simulink model "chaine_qpsk"  (R2023b)
settings: Solver=FixedStepDiscrete  StartTime=0.0  StopTime=(N/2 - 1)*2*Tb  FixedStep=2*Tb  RelTol=1e-3
values from neighbouring files (symbols this model uses):
  graine = P.graine    [parametres.m]    (also in parametres_perso.m = mod(sum(c .* (1:numel(c)) * 31) + 7 * numel(c), 2^31 - 1); partie2_1.m)
  N0 = Es / (2*g)    (= 0.158113883008)    [creer_qpsk.m]    (also in creer_qpsk_hamming.m = 0.276699295265; parametres.m = Eb / 10^(EbN0dB/10))
  Tb = 1    [parametres.m]    (also in partie2_1.m)
libraries: simulink x3
settings Model: Creator=e2507477  LastModifiedBy=e2507477

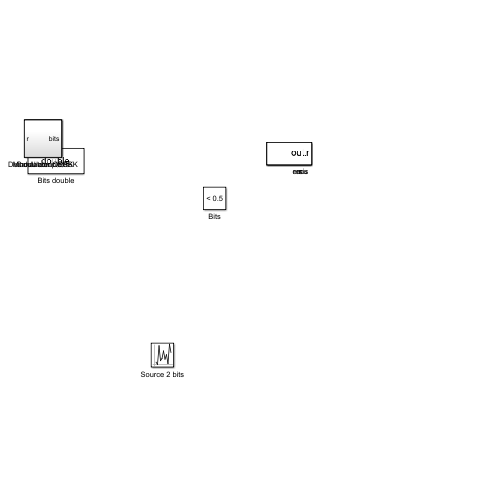
[thumbnail: Simulink's stored preview of the top-level diagram]
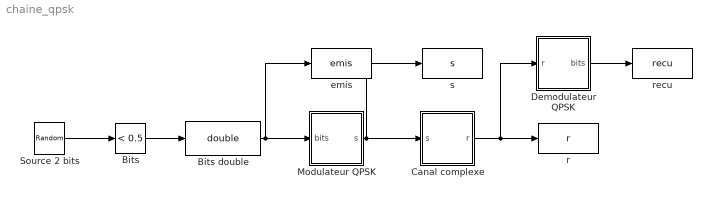
== system chaine_qpsk ==
  Bits : simulink/Logic and Bit Operations/Compare To Constant  relop=<  const=0.5  OutDataTypeStr=boolean
  Bits double : DataTypeConversion  OutDataTypeStr=double  SaturateOnIntegerOverflow=off  RndMeth=Floor
  Canal complexe : Subsystem
  Demodulateur QPSK : Subsystem
  Modulateur QPSK : Subsystem
  Source 2 bits : UniformRandomNumber  Minimum=zeros(1,2)  Maximum=ones(1,2)  Seed=round(graine) + 7919*(0:1)  SampleTime=2*Tb
  emis : ToWorkspace  VariableName=emis  SampleTime=-1
  r : ToWorkspace  VariableName=r  SampleTime=-1
  recu : ToWorkspace  VariableName=recu  SampleTime=-1
  s : ToWorkspace  VariableName=s  SampleTime=-1
  wires:
  Source 2 bits/1 -> Bits/1
  Bits/1 -> Bits double/1
  Bits double/1 -> Modulateur QPSK/1(bits), emis/1
  Modulateur QPSK/1(s) -> Canal complexe/1(s), s/1
  Canal complexe/1(r) -> Demodulateur QPSK/1(r), r/1
  Demodulateur QPSK/1(bits) -> recu/1

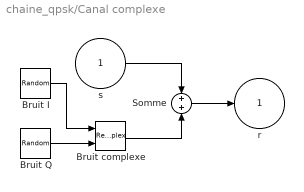
== system chaine_qpsk/Canal complexe ==
  s : Inport
  Bruit I : RandomNumber  Variance=N0/2  Seed=round(graine) + 50000  SampleTime=2*Tb
  Bruit Q : RandomNumber  Variance=N0/2  Seed=round(graine) + 60000  SampleTime=2*Tb
  Bruit complexe : RealImagToComplex
  Somme : Sum
  r : Outport
  wires:
  Somme/1 -> r/1
  Bruit complexe/1 -> Somme/2
  Bruit Q/1 -> Bruit complexe/2
  Bruit I/1 -> Bruit complexe/1
  s/1 -> Somme/1

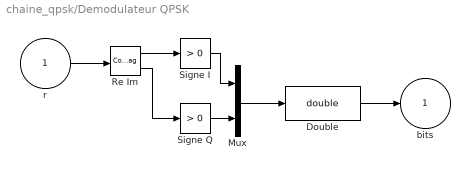
== system chaine_qpsk/Demodulateur QPSK ==
  r : Inport
  Double : DataTypeConversion  OutDataTypeStr=double  SaturateOnIntegerOverflow=off  RndMeth=Floor
  Mux : Mux  Inputs=2
  Re Im : ComplexToRealImag
  Signe I : simulink/Logic and Bit Operations/Compare To Constant  relop=>  const=0  OutDataTypeStr=boolean
  Signe Q : simulink/Logic and Bit Operations/Compare To Constant  relop=>  const=0  OutDataTypeStr=boolean
  bits : Outport
  wires:
  Double/1 -> bits/1
  Re Im/1 -> Signe I/1
  r/1 -> Re Im/1
  Mux/1 -> Double/1
  Signe Q/1 -> Mux/2
  Signe I/1 -> Mux/1
  Re Im/2 -> Signe Q/1

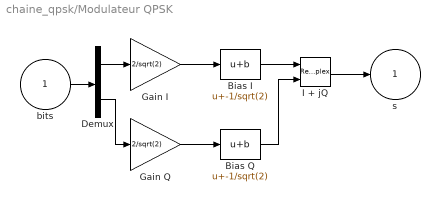
== system chaine_qpsk/Modulateur QPSK ==
  bits : Inport
  Bias I : Bias  Bias=-1/sqrt(2)  SaturateOnIntegerOverflow=off
  Bias Q : Bias  Bias=-1/sqrt(2)  SaturateOnIntegerOverflow=off
  Demux : Demux  Outputs=2
  Gain I : Gain  Gain=2/sqrt(2)
  Gain Q : Gain  Gain=2/sqrt(2)
  I + jQ : RealImagToComplex
  s : Outport
  wires:
  bits/1 -> Demux/1
  I + jQ/1 -> s/1
  Gain Q/1 -> Bias Q/1
  Gain I/1 -> Bias I/1
  Demux/1 -> Gain I/1
  Bias Q/1 -> I + jQ/2
  Bias I/1 -> I + jQ/1
  Demux/2 -> Gain Q/1
